simulink model "Pack_96S_Test"  (R2025b)
settings: Solver=FixedStepDiscrete  StartTime=0.0  StopTime=1  FixedStep=Ts  RelTol=1e-3
InitFcn:
  | init_BMS
undefined symbols (not defined in the file): Ts
libraries: BMS_Library x1
settings Model: Creator=Khadija  LastModifiedBy=Khadija

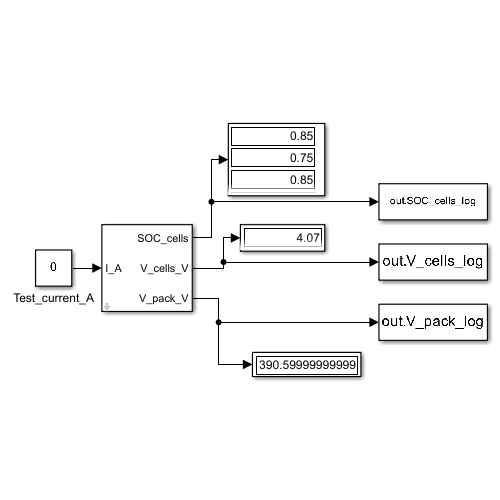
[thumbnail: Simulink's stored preview of the top-level diagram]
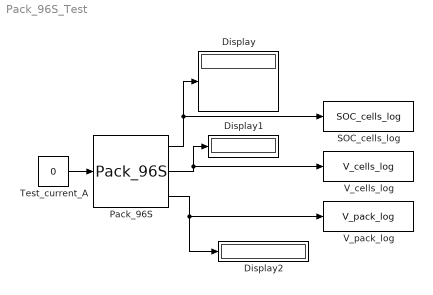
== system Pack_96S_Test ==
  Display : Display
  Display1 : Display
  Display2 : Display
  Pack_96S : BMS_Library/Pack_96S  SOC_init_pack=SOC0_pack
  SOC_cells_log : ToWorkspace  VariableName=SOC_cells_log  SaveFormat=Timeseries  SampleTime=-1
  Test_current_A : Constant  Value=0  SampleTime=Ts
  V_cells_log : ToWorkspace  VariableName=V_cells_log  SaveFormat=Timeseries  SampleTime=-1
  V_pack_log : ToWorkspace  VariableName=V_pack_log  SaveFormat=Timeseries  SampleTime=-1
  wires:
  Test_current_A/1 -> Pack_96S/1
  Pack_96S/1 -> Display/1, SOC_cells_log/1
  Pack_96S/2 -> V_cells_log/1, Display1/1
  Pack_96S/3 -> V_pack_log/1, Display2/1
